simulink model "hrg_wa_a4_physical_adapter"  (R2025a)
settings: Solver=FixedStepDiscrete  StartTime=0.0  StopTime=p.duration  FixedStep=p.Ts  RelTol=1e-3
model workspace (MAT data in the model file):
  c.detect = [-9972404109.88+545531236.399i  -249309643.885+13636860.8122i; 149494718.172-9008065.32861i  -10364964237.4+624623483.105i]
  c.sample_period_s = 2.5e-05
  c.drive = [1.0677844451e-06-2.20398878536e-07i  -3.17521469995e-08+7.37540079324e-09i; 2.13555769115e-08-4.4075121339e-09i  1.14308554761e-06-2.65485352229e-07i]
  c.nominal_detect = -9999678898.08+46914376.8426i
  c.frequency_Hz = 1000
  c.adapter.VFS = 1
  c.adapter.F0 = 1.1e-06
  c.adapter.M = [0.987525806615+0.203832884887i  0.0274313838571+0.00566131181148i; -0.0182507258254-0.00423917287679i  0.912549028973+0.211942495876i]
  c.adapter.matrix_codes = [64718 1798 -1196 59805 13358 371 -278 13890]
  c.adapter.profile = 'synthetic_independent_reference_only'
  c.adapter.phase_epoch = 's.phase before this sample update'
  p.schema = 'v10.1'
  p.synthetic = 1
  p.f0 = 1000
  p.gamma_intrinsic = 0.314159265359
  p.Cs = 1e-09
  p.G0 = 1e-10
  p.kappa = 1e-06
  p.b = 1.1e-06
  p.Cds = 0
  p.Rs = 1000
  p.B = 0.276990961962
  p.Omega = 0.5
  p.Ts = 2.5e-05
  p.Tc = 0.001
  p.duration = 0.8
  p.charge_target = 1e-11
  p.initial_fraction = 0.3
  p.theta0 = 0.4
  p.Cf = 1e-10
  p.Rf = 1000000000
  p.driver_tau = [2e-05; 2.4e-05]
  p.afe_bw = [20000; 18000]
  p.detect_matrix = [1  0.025; -0.015  1.04]
  p.drive_matrix = [1  -0.03; 0.02  1.08]
  p.split_hz = 0
  p.stiffness_axis = 0.37
  p.damping_half_difference = 0
  p.damping_axis = -0.23
  p.adc_span = 2
  p.adc_bits = 20
  p.dac_span = 2
  p.dac_bits = 18
  p.vmax = 1
  p.agc_bw = 5
  p.quad_bw = 4
  p.pll_gain = 30
  p.max_detune = 30
  p.virtual_rate = 0
  p.virtual_start_min_s = 0.25
  p.virtual_settle_fraction = 0.01
  p.predict_heading = 0
  p.max_heading_rate = 100
  p.virtual_validated_limit = 0.2
  p.min_amplitude_fraction = 0.02
  p.min_linearity = 0.1
  p.max_calibration_condition = 100
  p.max_frame_age = 0.002
  p.calibrate_detection = 1
  p.calibrate_drive = 1
  p.noise_rms_V = 0
  p.noise_seed = 20261030
  p.heading_start_s = 0
  p.zero_start_force = 1
  p.enable_tensor_ff = 0
  p.identified_dK = [0  0; 0  0]
  p.identified_dD = [0  0; 0  0]
  p.enable_iq_estimator = 0
  z.omega = [0.5 -0.5 0.25]
  z.x0 = [2.76318298201e-12; 1.16825502693e-12; 0; 0; 0; 0; 0; 0; 0; 0; 0; 0]
  z.segment = [1 1 1 1 1 1 1 1 1 1 1 1 ... (32001 elements, 32001x1)]
  z.Ad = [0.987688405123 5.68131323296e-08 -982.899001209 0.00680633562581 0 0 943869.866875 -6.2854468604 113668107.931 -505.246320907 62170953.3395 -882829.706009 ... (432 elements, 12x12x3)]
  z.Bd = reshape([1.07541978092e-16 2.15044631223e-18 1.17750014529e-11 2.35440509738e-13 0.71349520314 0 -1.10105605369e-08 -2.20157780066e-10 -9.65252715165e-07 -1.93016562843e-08 -4.58609339763e-07 -2.49830556256e-09 -2.80909408987e-18 1.01140599362e-16 -3.11685647158e-13 1.12226992357e-11 0 0.647133918541 2.90941885987e-10 -1.04757152027e-08 2.517993119e-08 -9.06591565342e-07 1.18833226824e-09 -4.18846719335e-07 1.07541962369e-16 2.15123249699e-18 1.1774999073e-11 2.3555950078e-13 0.71349520314 0 -1.10105584005e-08 -2.20264598683e-10 -9.65252579299e-07 -1.9308449605e-08 -4.58609353541e-07 -2.50098454879e-09 -2.80982753097e-18 1.01140578989e-16 -3.11797557364e-13 1.12226961271e-11 0 0.647133918541 2.91042214528e-10 -1.04757124158e-08 2.51862619997e-08 -9.06591389486e-07 1.19089244688e-09 -4.18846686132e-07 1.07541974162e-16 2.15064285844e-18 1.17750008581e-11 2.35470257502e-13 0.71349520314 0 -1.1010560003e-08 -2.20184484723e-10 -9.65252681206e-07 -1.93033546146e-08 -4.5860934321e-07 -2.49897530913e-09 -2.80927745017e-18 1.01140594269e-16 -3.11713624714e-13 1.12226984587e-11 0 0.647133918541 2.90966968126e-10 -1.04757145061e-08 2.51815138926e-08 -9.06591521385e-07 1.18897231291e-09 -4.18846711037e-07], [12 2 3])
  z.A = reshape([0 0 -39478417.6044 1.86264514923e-09 0 0 0 0 0 0 0 0 0 0 -1.86264514923e-09 -39478417.6044 0 0 0 0 0 0 0 0 1 0 -0.628318530718 -0.553981923923 0 0 -1000000000 0 0 0 0 0 0 1 0.553981923923 -0.628318530718 0 0 0 -1000000000 0 0 0 0 0 0 1.1e-06 2.2e-08 -50000 0 0 0 0 0 0 0 0 0 -3.3e-08 1.188e-06 0 -41666.6666667 0 0 0 0 0 0 0 0 1e-06 0 0 0 -1000000.1 0 10000000 0 0 0 0 0 0 1e-06 0 0 0 -1000000.1 0 10000000 0 0 0 0 0 0 0 0 0 0 -10 0 125663.706144 -1696.46003294 0 0 0 0 0 0 0 0 0 -10 3141.59265359 117621.22895 0 0 0 0 0 0 0 0 0 0 -125663.706144 0 0 0 0 0 0 0 0 0 0 0 0 -113097.335529 0 0 -39478417.6044 1.86264514923e-09 0 0 0 0 0 0 0 0 0 0 -1.86264514923e-09 -39478417.6044 0 0 0 0 0 0 0 0 1 0 -0.628318530718 0.553981923923 0 0 -1000000000 0 0 0 0 0 0 1 -0.553981923923 -0.628318530718 0 0 0 -1000000000 0 0 0 0 0 0 1.1e-06 2.2e-08 -50000 0 0 0 0 0 0 0 0 0 -3.3e-08 1.188e-06 0 -41666.6666667 0 0 0 0 0 0 0 0 1e-06 0 0 0 -1000000.1 0 10000000 0 0 0 0 0 0 1e-06 0 0 0 -1000000.1 0 10000000 0 0 0 0 0 0 0 0 0 0 -10 0 125663.706144 -1696.46003294 0 0 0 0 0 0 0 0 0 -10 3141.59265359 117621.22895 0 0 0 0 0 0 0 0 0 0 -125663.706144 0 0 0 0 0 0 0 0 0 0 0 0 -113097.335529 0 0 -39478417.6044 1.86264514923e-09 0 0 0 0 0 0 0 0 0 0 -1.86264514923e-09 -39478417.6044 0 0 0 0 0 0 0 0 1 0 -0.628318530718 -0.276990961962 0 0 -1000000000 0 0 0 0 0 0 1 0.276990961962 -0.628318530718 0 0 0 -1000000000 0 0 0 0 0 0 1.1e-06 2.2e-08 -50000 0 0 0 0 0 0 0 0 0 -3.3e-08 1.188e-06 0 -41666.6666667 0 0 0 0 0 0 0 0 1e-06 0 0 0 -1000000.1 0 10000000 0 0 0 0 0 0 1e-06 0 0 0 -1000000.1 0 10000000 0 0 0 0 0 0 0 0 0 0 -10 0 125663.706144 -1696.46003294 0 0 0 0 0 0 0 0 0 -10 3141.59265359 117621.22895 0 0 0 0 0 0 0 0 0 0 -125663.706144 0 0 0 0 0 0 0 0 0 0 0 0 -113097.335529], [12 12 3])
  z.B = reshape([0 0 0 0 50000 0 0 0 0 0 0 0 0 0 0 0 0 41666.6666667 0 0 0 0 0 0 0 0 0 0 50000 0 0 0 0 0 0 0 0 0 0 0 0 41666.6666667 0 0 0 0 0 0 0 0 0 0 50000 0 0 0 0 0 0 0 0 0 0 0 0 41666.6666667 0 0 0 0 0 0], [12 2 3])
  z.noise = [0 0 0 0 0 0 0 0 0 0 0 0 ... (64002 elements, 32001x2)]
settings Model: Creator=11725  LastModifiedBy=11725

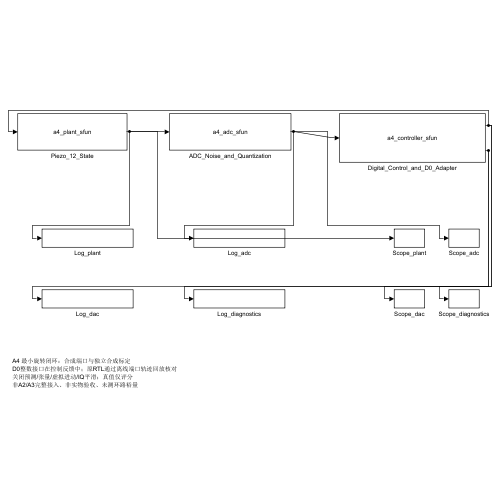
[thumbnail: Simulink's stored preview of the top-level diagram]
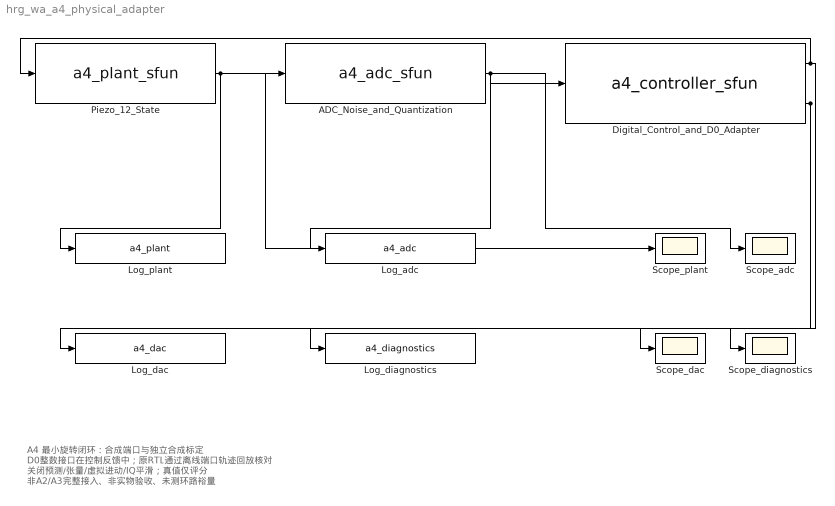
== system hrg_wa_a4_physical_adapter ==
  note: A4 最小旋转闭环：合成端口与独立合成标定
      | D0整数接口在控制反馈中；原RTL通过离线端口轨迹回放核对
      | 关闭预测/张量/虚拟进动/IQ平滑；真值仅评分
      | 非A2/A3完整接入、非实物验收、未测环路裕量
  ADC_Noise_and_Quantization : M-S-Function  FunctionName=a4_adc_sfun  Parameters=p,z
  Digital_Control_and_D0_Adapter : M-S-Function  FunctionName=a4_controller_sfun  Parameters=p,c
  Log_adc : ToWorkspace  VariableName=a4_adc  SaveFormat=Timeseries  SampleTime=-1
  Log_dac : ToWorkspace  VariableName=a4_dac  SaveFormat=Timeseries  SampleTime=-1
  Log_diagnostics : ToWorkspace  VariableName=a4_diagnostics  SaveFormat=Timeseries  SampleTime=-1
  Log_plant : ToWorkspace  VariableName=a4_plant  SaveFormat=Timeseries  SampleTime=-1
  Piezo_12_State : M-S-Function  FunctionName=a4_plant_sfun  Parameters=p,z
  Scope_adc : Scope
  Scope_dac : Scope
  Scope_diagnostics : Scope
  Scope_plant : Scope
  wires:
  Piezo_12_State/1 -> ADC_Noise_and_Quantization/1, Log_plant/1, Scope_plant/1
  ADC_Noise_and_Quantization/1 -> Digital_Control_and_D0_Adapter/1, Log_adc/1, Scope_adc/1
  Digital_Control_and_D0_Adapter/1 -> Piezo_12_State/1, Log_dac/1, Scope_dac/1
  Digital_Control_and_D0_Adapter/2 -> Log_diagnostics/1, Scope_diagnostics/1
